simulink model "T8electromec"  (R2024b)
settings: Solver=VariableStepAuto  StartTime=0.0  StopTime=10.0  RelTol=1e-3
InitFcn:
  |     Ra=2;
  |     Kt=0.01;
  |     b=0.0012;
  |     La=0.023;
  |     Ke=0.01;
  |     J=0.001;
  |     V=5;
settings Model: Creator=sanch

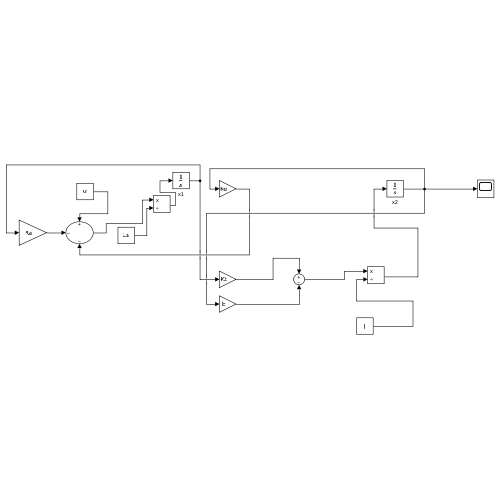
[thumbnail: Simulink's stored preview of the top-level diagram]
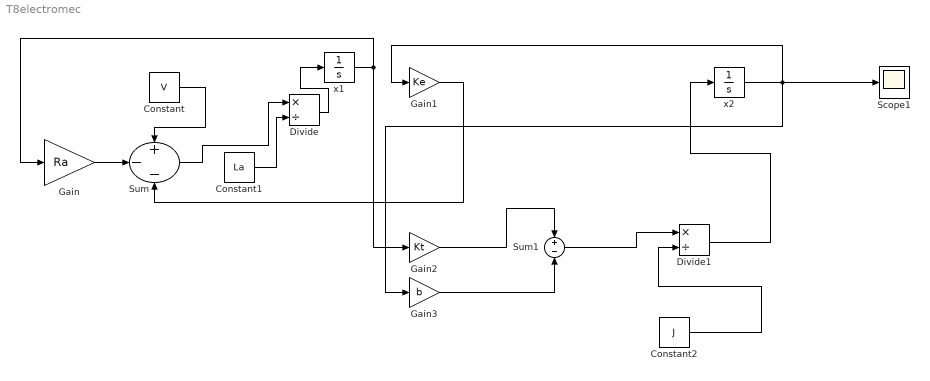
== system T8electromec ==
  Constant : Constant  Value=V
  Constant1 : Constant  Value=La
  Constant2 : Constant  Value=J
  Divide : Product  Inputs=*/
  Divide1 : Product  Inputs=*/
  Gain : Gain  Gain=Ra
  Gain1 : Gain  Gain=Ke
  Gain2 : Gain  Gain=Kt
  Gain3 : Gain  Gain=b
  Scope1 : Scope
  Sum : Sum  Inputs=+--
  Sum1 : Sum  Inputs=+-
  x1 : Integrator
  x2 : Integrator
  wires:
  Constant/1 -> Sum/1
  Gain/1 -> Sum/2
  Gain1/1 -> Sum/3
  Sum/1 -> Divide/1
  Constant1/1 -> Divide/2
  Divide/1 -> x1/1
  x1/1 -> Gain/1, Gain2/1
  x2/1 -> Gain3/1, Scope1/1, Gain1/1
  Gain2/1 -> Sum1/1
  Gain3/1 -> Sum1/2
  Sum1/1 -> Divide1/1
  Constant2/1 -> Divide1/2
  Divide1/1 -> x2/1
